simulink model "copia 15_10_26"  (R2026a)
settings: Solver=VariableStepAuto  StopTime=10  RelTol=1e-2  AbsTol=1e-2  EnableMultiTasking=on
values from neighbouring files (symbols this model uses):
  effective_bulkmodulus = 750e6    (= 750000000)    [MARLUP_hydr_params.m]
  m_load = 20    [MARLUP_hydr_params.m]
  p_supply = 160e5    (= 16000000)    [MARLUP_hydr_params.m]
  p_tank = 1.01325e5    (= 101325)    [MARLUP_hydr_params.m]
undefined symbols (not defined in the file or in its folder): cyl, Kd_heave, Kd_pitch, Kd_roll, Ki_heave, Ki_pitch, Ki_roll, Kp_heave, Kp_pitch, Kp_roll, pipe, Tinv, Ts, valve, X, Y, Z
libraries: sm_lib x75, nesl_utility x14, slpidlib x6, simulink x3
(part 5 of 5)

== system copia 15_10_26/PLANTA/Actuador_Hidraulico_2/cylinder_63_36/volume A chamber ==
  note: ∆𝑉 = −𝑉0 / 𝐵𝑛 ∗ ∆𝑝
  Q_in : Inport
  " dV/dt" : Inport  Port=2
  " V" : Inport  Port=3
  " B" : Inport  Port=4
  Integrator : Integrator  InitialCondition=cyl.p0A  AbsoluteTolerance=10
  Product : Product  Inputs=*/*  InputSameDT=on  SaturateOnIntegerOverflow=on  OutDataTypeStr=Inherit: Same as first input
  Saturation : Saturate  UpperLimit=inf  LowerLimit=-1e5
  Sum1 : Sum  Inputs=+-  InputSameDT=on  SaturateOnIntegerOverflow=on  OutDataTypeStr=Inherit: Same as first input
  p : Outport  VectorParamsAs1DForOutWhenUnconnected=off
  wires:
  Integrator/1 -> Saturation/1
  Product/1 -> Integrator/1
  Sum1/1 -> Product/1
  " B"/1 -> Product/3
  Saturation/1 -> p/1
  Q_in/1 -> Sum1/1
  " V"/1 -> Product/2
  " dV/dt"/1 -> Sum1/2

== system copia 15_10_26/PLANTA/Actuador_Hidraulico_2/cylinder_63_36/volume B chamber ==
  Q_in : Inport
  " dV/dt" : Inport  Port=2
  " V" : Inport  Port=3
  " B" : Inport  Port=4
  Integrator : Integrator  InitialCondition=cyl.p0B  AbsoluteTolerance=10
  Product : Product  Inputs=*/*  InputSameDT=on  SaturateOnIntegerOverflow=on  OutDataTypeStr=Inherit: Same as first input
  Saturation : Saturate  UpperLimit=inf  LowerLimit=-1e5
  Sum1 : Sum  Inputs=+-  InputSameDT=on  SaturateOnIntegerOverflow=on  OutDataTypeStr=Inherit: Same as first input
  p : Outport  VectorParamsAs1DForOutWhenUnconnected=off
  wires:
  " dV/dt"/1 -> Sum1/2
  " V"/1 -> Product/2
  Q_in/1 -> Sum1/1
  Saturation/1 -> p/1
  " B"/1 -> Product/3
  Sum1/1 -> Product/1
  Product/1 -> Integrator/1
  Integrator/1 -> Saturation/1

== system copia 15_10_26/PLANTA/Actuador_Hidraulico_2/gate_load_mass/load_fric ==
  v : Inport
  Gain1 : Gain  Gain=-1
  Product : Product  Inputs=4
  Sign : Signum
  coeff_fric : Constant  Value=0.7e5
  F_fric_load : Outport  VectorParamsAs1DForOutWhenUnconnected=off
  wires:
  Product/1 -> F_fric_load/1
  Sign/1 -> Gain1/1
  coeff_fric/1 -> Product/4
  Gain1/1 -> Product/1
  v/1 -> Product/2, Product/3, Sign/1

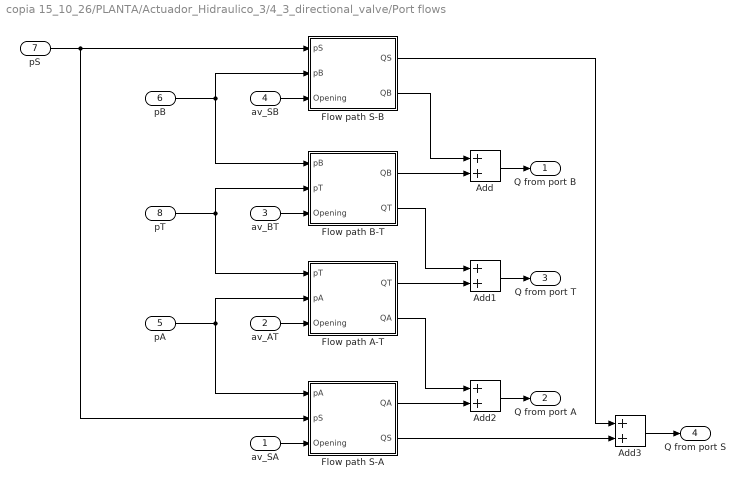
== system copia 15_10_26/PLANTA/Actuador_Hidraulico_3/4_3_directional_valve/Port flows ==
  av_SA : Inport
  av_AT : Inport  Port=2
  av_BT : Inport  Port=3
  av_SB : Inport  Port=4
  pA : Inport  Port=5
  pB : Inport  Port=6
  pS : Inport  Port=7
  pT : Inport  Port=8
  Add{,1..3} (4 alike) : Sum
  Flow path A-T : Subsystem  mask(Hydraulic){DPN=valve.dpN, QN=valve.QN, ptr=valve.ptr}
      mask prompts: DPN "Nominal Pressure Difference [Pa] :"; QN "Flow at nominal pressure difference and maximum opening [m^3/s] :"; ptr "Transition pressure [Pa] :"
      mask help:
      | Implements numerically robust turbulent flow equation. Polynomial flow equation is
      | used when abs(dp) is smaller than transition pressure.
      | [Source: Ellman, A. & Piche, R. 1996.
      | A Modified Orifice Flow Formula for Numerical Simulation of Fluid Power Systems.
      | Fluid Power Systems and Technology, ASME]
      mask init:
      | K = QN/(sqrt(DPN));
  Flow path B-T : Subsystem  mask(Hydraulic){DPN=valve.dpN, QN=valve.QN, ptr=valve.ptr}
      mask prompts: DPN "Nominal Pressure Difference [Pa] :"; QN "Flow at nominal pressure difference and maximum opening [m^3/s] :"; ptr "Transition pressure [Pa] :"
      mask help:
      | Implements numerically robust turbulent flow equation. Polynomial flow equation is
      | used when abs(dp) is smaller than transition pressure.
      | [Source: Ellman, A. & Piche, R. 1996.
      | A Modified Orifice Flow Formula for Numerical Simulation of Fluid Power Systems.
      | Fluid Power Systems and Technology, ASME]
      mask init:
      | K = QN/(sqrt(DPN));
  Flow path S-A : Subsystem  mask(Hydraulic){DPN=valve.dpN, QN=valve.QN, ptr=valve.ptr}
      mask prompts: DPN "Nominal Pressure Difference [Pa] :"; QN "Flow at nominal pressure difference and maximum opening [m^3/s] :"; ptr "Transition pressure [Pa] :"
      mask help:
      | Implements numerically robust turbulent flow equation. Polynomial flow equation is
      | used when abs(dp) is smaller than transition pressure.
      | [Source: Ellman, A. & Piche, R. 1996.
      | A Modified Orifice Flow Formula for Numerical Simulation of Fluid Power Systems.
      | Fluid Power Systems and Technology, ASME]
      mask init:
      | K = QN/(sqrt(DPN));
  Flow path S-B : Subsystem  mask(Hydraulic){DPN=valve.dpN, QN=valve.QN, ptr=valve.ptr}
      mask prompts: DPN "Nominal Pressure Difference [Pa] :"; QN "Flow at nominal pressure difference and maximum opening [m^3/s] :"; ptr "Transition pressure [Pa] :"
      mask help:
      | Implements numerically robust turbulent flow equation. Polynomial flow equation is
      | used when abs(dp) is smaller than transition pressure.
      | [Source: Ellman, A. & Piche, R. 1996.
      | A Modified Orifice Flow Formula for Numerical Simulation of Fluid Power Systems.
      | Fluid Power Systems and Technology, ASME]
      mask init:
      | K = QN/(sqrt(DPN));
  Q from port B : Outport  VectorParamsAs1DForOutWhenUnconnected=off
  Q from port A : Outport  Port=2  VectorParamsAs1DForOutWhenUnconnected=off
  Q from port T : Outport  Port=3  VectorParamsAs1DForOutWhenUnconnected=off
  Q from port S : Outport  Port=4  VectorParamsAs1DForOutWhenUnconnected=off
  wires:
  av_SA/1 -> Flow path S-A/3(Opening)
  av_AT/1 -> Flow path A-T/3(Opening)
  av_BT/1 -> Flow path B-T/3(Opening)
  pA/1 -> Flow path A-T/2(pA), Flow path S-A/1(pA)
  pB/1 -> Flow path B-T/1(pB), Flow path S-B/2(pB)
  pS/1 -> Flow path S-B/1(pS), Flow path S-A/2(pS)
  pT/1 -> Flow path A-T/1(pT), Flow path B-T/2(pT)
  Add/1 -> Q from port B/1
  Add1/1 -> Q from port T/1
  Add2/1 -> Q from port A/1
  Add3/1 -> Q from port S/1
  Flow path S-B/1(QS) -> Add3/1
  Flow path S-A/2(QS) -> Add3/2
  Flow path S-A/1(QA) -> Add2/2
  Flow path A-T/2(QA) -> Add2/1
  Flow path A-T/1(QT) -> Add1/2
  Flow path B-T/2(QT) -> Add1/1
  Flow path B-T/1(QB) -> Add/2
  Flow path S-B/2(QB) -> Add/1
  av_SB/1 -> Flow path S-B/3(Opening)

== system copia 15_10_26/PLANTA/Actuador_Hidraulico_3/4_3_directional_valve/Relative opening of flow paths ==
  x : Inport
  Gain : Gain  Gain=-1
  Lookup Table5 : Lookup  InputValues=[0.01 0.05 0.1 0.2 0.3 0.4 1]  Table=[0.01 0.039 0.078 0.16 0.23 0.31 0.78]  SaturateOnIntegerOverflow=off
  Lookup Table6 : Lookup  InputValues=[0.01 0.05 0.1 0.2 0.3 0.4 1]  Table=[0.01 0.036 0.072 0.14 0.22 0.29 0.72]  SaturateOnIntegerOverflow=off
  Lookup Table7 : Lookup  InputValues=[0.01 0.05 0.1 0.2 0.3 0.4 1]  Table=[0.01 0.039 0.077 0.15 0.23 0.31 0.77]  SaturateOnIntegerOverflow=off
  Lookup Table8 : Lookup  InputValues=[0.01 0.05 0.1 0.2 0.3 0.4 1]  Table=[0.01 0.035 0.070 0.14 0.21 0.28 0.70]  SaturateOnIntegerOverflow=off
  Saturation1 : Saturate  UpperLimit=1  LowerLimit=0
  Saturation2 : Saturate  UpperLimit=0  LowerLimit=-1
  av_SA : Outport  VectorParamsAs1DForOutWhenUnconnected=off
  av_AT : Outport  Port=2  VectorParamsAs1DForOutWhenUnconnected=off
  av_BT : Outport  Port=3  VectorParamsAs1DForOutWhenUnconnected=off
  av_SB : Outport  Port=4  VectorParamsAs1DForOutWhenUnconnected=off
  wires:
  x/1 -> Saturation2/1, Saturation1/1
  Saturation2/1 -> Gain/1
  Lookup Table8/1 -> av_AT/1
  Lookup Table7/1 -> av_SB/1
  Lookup Table6/1 -> av_BT/1
  Lookup Table5/1 -> av_SA/1
  Saturation1/1 -> Lookup Table5/1, Lookup Table6/1
  Gain/1 -> Lookup Table8/1, Lookup Table7/1

== system copia 15_10_26/PLANTA/Actuador_Hidraulico_3/4_3_directional_valve/Valve dynamics ==
  u : Inport
  Rate Limiter : RateLimiter  RisingSlewLimit=valve.ratelimit  FallingSlewLimit=-valve.ratelimit  SampleTimeMode=inherited
  Saturation limits [-1,1] : Saturate  UpperLimit=1  LowerLimit=-1
  Saturation limits [-1,1]2 : Saturate  UpperLimit=1  LowerLimit=-1
  Transfer Fcn1 : TransferFcn  Denominator=[valve.tau 1]
  Transport Delay of the valve : TransportDelay  DelayTime=valve.delay
  x : Outport  VectorParamsAs1DForOutWhenUnconnected=off
  wires:
  Saturation limits [-1,1]/1 -> Transport Delay of the valve/1
  Transport Delay of the valve/1 -> Rate Limiter/1
  Rate Limiter/1 -> Transfer Fcn1/1
  u/1 -> Saturation limits [-1,1]/1
  Transfer Fcn1/1 -> Saturation limits [-1,1]2/1
  Saturation limits [-1,1]2/1 -> x/1

== system copia 15_10_26/PLANTA/Actuador_Hidraulico_3/cylinder_63_36/A-chamber and pipe size submodel ==
  x_cyl : Inport
  A : Gain  Gain=pipe.area
  A chamber dead volume : Constant  Value=cyl.V0A
  Add : Sum  Inputs=+++
  Gain : Gain  Gain=cyl.A_piston
  Lenght : Constant  Value=pipe.lenght
  V : Outport  VectorParamsAs1DForOutWhenUnconnected=off
  wires:
  A/1 -> Add/3
  Lenght/1 -> A/1
  A chamber dead volume/1 -> Add/2
  Gain/1 -> Add/1
  x_cyl/1 -> Gain/1
  Add/1 -> V/1

== system copia 15_10_26/PLANTA/Actuador_Hidraulico_3/cylinder_63_36/B-chamber and pipe size submodel ==
  x_cyl : Inport
  A : Gain  Gain=pipe.area
  Add : Sum  Inputs=+-
  Add1 : Sum  Inputs=+++
  B chamber dead volume : Constant  Value=cyl.V0B
  Cylinder stroke : Constant  Value=cyl.stroke
  Gain1 : Gain  Gain=cyl.A_rodside
  Lenght : Constant  Value=pipe.lenght
  V : Outport  VectorParamsAs1DForOutWhenUnconnected=off
  wires:
  A/1 -> Add1/3
  Lenght/1 -> A/1
  Cylinder stroke/1 -> Add/1
  Gain1/1 -> Add1/1
  Add/1 -> Gain1/1
  x_cyl/1 -> Add/2
  B chamber dead volume/1 -> Add1/2
  Add1/1 -> V/1

== system copia 15_10_26/PLANTA/Actuador_Hidraulico_3/cylinder_63_36/dynamic_fric_limited ==
  v : Inport
  Abs : Abs  SaturateOnIntegerOverflow=off
  Product : Product
  Sign : Signum
  cyl_fric_up_to_100mm/s : Lookup_n-D  NumberOfTableDimensions=1  BreakpointsForDimension1=|  Table=|  InternalRulePriority=Speed  RndMeth=Simplest
      BreakpointsForDimension1=|
      | [0
      | 5
      | 10
      | 15
      | 20
      | 25
      | 30
      | 35
      | 40
      | 45
      | 50
      | 55
      | 60
      | 65
      | 70
      | 75
      | 80
      | 85
      | 90
      | 95
      | 100]./1e3;
      Table=|
      | [0
      | 242
      | 550
      | 838
      | 996
      | 972
      | 850
      | 757
      | 728
      | 733
      | 744
      | 753
      | 759
      | 765
      | 770
      | 775
      | 780
      | 785
      | 790
      | 795
      | 800];
  F_fric : Outport  VectorParamsAs1DForOutWhenUnconnected=off
  wires:
  Abs/1 -> cyl_fric_up_to_100mm/s/1
  v/1 -> Sign/1, Abs/1
  cyl_fric_up_to_100mm/s/1 -> Product/1
  Sign/1 -> Product/2
  Product/1 -> F_fric/1

== system copia 15_10_26/PLANTA/Actuador_Hidraulico_3/cylinder_63_36/volume A chamber ==
  note: ∆𝑉 = −𝑉0 / 𝐵𝑛 ∗ ∆𝑝
  Q_in : Inport
  " dV/dt" : Inport  Port=2
  " V" : Inport  Port=3
  " B" : Inport  Port=4
  Integrator : Integrator  InitialCondition=cyl.p0A  AbsoluteTolerance=10
  Product : Product  Inputs=*/*  InputSameDT=on  SaturateOnIntegerOverflow=on  OutDataTypeStr=Inherit: Same as first input
  Saturation : Saturate  UpperLimit=inf  LowerLimit=-1e5
  Sum1 : Sum  Inputs=+-  InputSameDT=on  SaturateOnIntegerOverflow=on  OutDataTypeStr=Inherit: Same as first input
  p : Outport  VectorParamsAs1DForOutWhenUnconnected=off
  wires:
  Integrator/1 -> Saturation/1
  Product/1 -> Integrator/1
  Sum1/1 -> Product/1
  " B"/1 -> Product/3
  Saturation/1 -> p/1
  Q_in/1 -> Sum1/1
  " V"/1 -> Product/2
  " dV/dt"/1 -> Sum1/2

== system copia 15_10_26/PLANTA/Actuador_Hidraulico_3/cylinder_63_36/volume B chamber ==
  Q_in : Inport
  " dV/dt" : Inport  Port=2
  " V" : Inport  Port=3
  " B" : Inport  Port=4
  Integrator : Integrator  InitialCondition=cyl.p0B  AbsoluteTolerance=10
  Product : Product  Inputs=*/*  InputSameDT=on  SaturateOnIntegerOverflow=on  OutDataTypeStr=Inherit: Same as first input
  Saturation : Saturate  UpperLimit=inf  LowerLimit=-1e5
  Sum1 : Sum  Inputs=+-  InputSameDT=on  SaturateOnIntegerOverflow=on  OutDataTypeStr=Inherit: Same as first input
  p : Outport  VectorParamsAs1DForOutWhenUnconnected=off
  wires:
  " dV/dt"/1 -> Sum1/2
  " V"/1 -> Product/2
  Q_in/1 -> Sum1/1
  Saturation/1 -> p/1
  " B"/1 -> Product/3
  Sum1/1 -> Product/1
  Product/1 -> Integrator/1
  Integrator/1 -> Saturation/1

== system copia 15_10_26/PLANTA/Actuador_Hidraulico_3/gate_load_mass/load_fric ==
  v : Inport
  Gain1 : Gain  Gain=-1
  Product : Product  Inputs=4
  Sign : Signum
  coeff_fric : Constant  Value=0.7e5
  F_fric_load : Outport  VectorParamsAs1DForOutWhenUnconnected=off
  wires:
  Product/1 -> F_fric_load/1
  Sign/1 -> Gain1/1
  coeff_fric/1 -> Product/4
  Gain1/1 -> Product/1
  v/1 -> Product/2, Product/3, Sign/1

== system copia 15_10_26/PLANTA/Actuador_Hidraulico_1/4_3_directional_valve/Port flows/Flow path A-T ==
  pT : Inport
  pA : Inport  Port=2
  Opening : Inport  Port=3
  Abs : Abs  ZeroCross=off
  Flow coefficient : Gain  Gain=K  SaturateOnIntegerOverflow=on  OutDataTypeStr=Inherit: Same as input  ParamDataTypeStr=Inherit: Same as input
  Gain1 : Gain  Gain=-1  SaturateOnIntegerOverflow=on  OutDataTypeStr=Inherit: Same as input  ParamDataTypeStr=Inherit: Same as input
  Limit opening to non-negative : Saturate  UpperLimit=inf  LowerLimit=0
  Math Function1 : Math  Operator=sqrt  SignedPower=on
  Mux : Mux  Inputs=2
  Polynomial flow equation : Fcn  Expr=u[2]*u[1]/2.0/sqrt(ptr)*(3-u[1]/ptr)
  Product : Product  InputSameDT=on  SaturateOnIntegerOverflow=on  OutDataTypeStr=Inherit: Same as first input
  Product1 : Product  InputSameDT=on  SaturateOnIntegerOverflow=on  OutDataTypeStr=Inherit: Same as first input
  Sign : Signum  ZeroCross=off
  Sum : Sum  Inputs=|+-
  Switch : Switch  Threshold=ptr  ZeroCross=off
  QT : Outport  InitialOutput=0  VectorParamsAs1DForOutWhenUnconnected=off
  QA : Outport  Port=2  InitialOutput=0  VectorParamsAs1DForOutWhenUnconnected=off
  wires:
  Opening/1 -> Limit opening to non-negative/1
  Sum/1 -> Abs/1, Sign/1
  Polynomial flow equation/1 -> Switch/3
  Mux/1 -> Polynomial flow equation/1
  Product/1 -> Switch/1
  Math Function1/1 -> Product/1
  Abs/1 -> Mux/1, Switch/2, Math Function1/1
  Limit opening to non-negative/1 -> Flow coefficient/1
  Flow coefficient/1 -> Product/2, Mux/2
  Sign/1 -> Product1/1
  Product1/1 -> Gain1/1, QT/1
  Switch/1 -> Product1/2
  pA/1 -> Sum/1
  pT/1 -> Sum/2
  Gain1/1 -> QA/1

== system copia 15_10_26/PLANTA/Actuador_Hidraulico_1/4_3_directional_valve/Port flows/Flow path B-T ==
  pB : Inport
  pT : Inport  Port=2
  Opening : Inport  Port=3
  Abs : Abs  ZeroCross=off
  Flow coefficient : Gain  Gain=K  SaturateOnIntegerOverflow=on  OutDataTypeStr=Inherit: Same as input  ParamDataTypeStr=Inherit: Same as input
  Gain1 : Gain  Gain=-1  SaturateOnIntegerOverflow=on  OutDataTypeStr=Inherit: Same as input  ParamDataTypeStr=Inherit: Same as input
  Limit opening to non-negative : Saturate  UpperLimit=inf  LowerLimit=0
  Math Function1 : Math  Operator=sqrt  SignedPower=on
  Mux : Mux  Inputs=2
  Polynomial flow equation : Fcn  Expr=u[2]*u[1]/2.0/sqrt(ptr)*(3-u[1]/ptr)
  Product : Product  InputSameDT=on  SaturateOnIntegerOverflow=on  OutDataTypeStr=Inherit: Same as first input
  Product1 : Product  InputSameDT=on  SaturateOnIntegerOverflow=on  OutDataTypeStr=Inherit: Same as first input
  Sign : Signum  ZeroCross=off
  Sum : Sum  Inputs=|+-
  Switch : Switch  Threshold=ptr  ZeroCross=off
  QB : Outport  InitialOutput=0  VectorParamsAs1DForOutWhenUnconnected=off
  QT : Outport  Port=2  InitialOutput=0  VectorParamsAs1DForOutWhenUnconnected=off
  wires:
  Gain1/1 -> QB/1
  pT/1 -> Sum/2
  pB/1 -> Sum/1
  Switch/1 -> Product1/2
  Product1/1 -> QT/1, Gain1/1
  Sign/1 -> Product1/1
  Flow coefficient/1 -> Mux/2, Product/2
  Limit opening to non-negative/1 -> Flow coefficient/1
  Abs/1 -> Math Function1/1, Switch/2, Mux/1
  Math Function1/1 -> Product/1
  Product/1 -> Switch/1
  Mux/1 -> Polynomial flow equation/1
  Polynomial flow equation/1 -> Switch/3
  Sum/1 -> Sign/1, Abs/1
  Opening/1 -> Limit opening to non-negative/1

== system copia 15_10_26/PLANTA/Actuador_Hidraulico_1/4_3_directional_valve/Port flows/Flow path S-A ==
  pA : Inport
  pS : Inport  Port=2
  Opening : Inport  Port=3
  Abs : Abs  ZeroCross=off
  Flow coefficient : Gain  Gain=K  SaturateOnIntegerOverflow=on  OutDataTypeStr=Inherit: Same as input  ParamDataTypeStr=Inherit: Same as input
  Gain1 : Gain  Gain=-1  SaturateOnIntegerOverflow=on  OutDataTypeStr=Inherit: Same as input  ParamDataTypeStr=Inherit: Same as input
  Limit opening to non-negative : Saturate  UpperLimit=inf  LowerLimit=0
  Math Function1 : Math  Operator=sqrt  SignedPower=on
  Mux : Mux  Inputs=2
  Polynomial flow equation : Fcn  Expr=u[2]*u[1]/2.0/sqrt(ptr)*(3-u[1]/ptr)
  Product : Product  InputSameDT=on  SaturateOnIntegerOverflow=on  OutDataTypeStr=Inherit: Same as first input
  Product1 : Product  InputSameDT=on  SaturateOnIntegerOverflow=on  OutDataTypeStr=Inherit: Same as first input
  Sign : Signum  ZeroCross=off
  Sum : Sum  Inputs=|+-
  Switch : Switch  Threshold=ptr  ZeroCross=off
  QA : Outport  InitialOutput=0  VectorParamsAs1DForOutWhenUnconnected=off
  QS : Outport  Port=2  InitialOutput=0  VectorParamsAs1DForOutWhenUnconnected=off
  wires:
  Opening/1 -> Limit opening to non-negative/1
  Sum/1 -> Abs/1, Sign/1
  Polynomial flow equation/1 -> Switch/3
  Mux/1 -> Polynomial flow equation/1
  Product/1 -> Switch/1
  Math Function1/1 -> Product/1
  Abs/1 -> Mux/1, Switch/2, Math Function1/1
  Limit opening to non-negative/1 -> Flow coefficient/1
  Flow coefficient/1 -> Product/2, Mux/2
  Sign/1 -> Product1/1
  Product1/1 -> Gain1/1, QA/1
  Switch/1 -> Product1/2
  pS/1 -> Sum/1
  pA/1 -> Sum/2
  Gain1/1 -> QS/1

== system copia 15_10_26/PLANTA/Actuador_Hidraulico_1/4_3_directional_valve/Port flows/Flow path S-B ==
  pS : Inport
  pB : Inport  Port=2
  Opening : Inport  Port=3
  Abs : Abs  ZeroCross=off
  Flow coefficient : Gain  Gain=K  SaturateOnIntegerOverflow=on  OutDataTypeStr=Inherit: Same as input  ParamDataTypeStr=Inherit: Same as input
  Gain1 : Gain  Gain=-1  SaturateOnIntegerOverflow=on  OutDataTypeStr=Inherit: Same as input  ParamDataTypeStr=Inherit: Same as input
  Limit opening to non-negative : Saturate  UpperLimit=inf  LowerLimit=0
  Math Function1 : Math  Operator=sqrt  SignedPower=on
  Mux : Mux  Inputs=2
  Polynomial flow equation : Fcn  Expr=u[2]*u[1]/2.0/sqrt(ptr)*(3-u[1]/ptr)
  Product : Product  InputSameDT=on  SaturateOnIntegerOverflow=on  OutDataTypeStr=Inherit: Same as first input
  Product1 : Product  InputSameDT=on  SaturateOnIntegerOverflow=on  OutDataTypeStr=Inherit: Same as first input
  Sign : Signum  ZeroCross=off
  Sum : Sum  Inputs=|+-
  Switch : Switch  Threshold=ptr  ZeroCross=off
  QS : Outport  InitialOutput=0  VectorParamsAs1DForOutWhenUnconnected=off
  QB : Outport  Port=2  InitialOutput=0  VectorParamsAs1DForOutWhenUnconnected=off
  wires:
  Gain1/1 -> QS/1
  pB/1 -> Sum/2
  pS/1 -> Sum/1
  Switch/1 -> Product1/2
  Product1/1 -> QB/1, Gain1/1
  Sign/1 -> Product1/1
  Flow coefficient/1 -> Mux/2, Product/2
  Limit opening to non-negative/1 -> Flow coefficient/1
  Abs/1 -> Math Function1/1, Switch/2, Mux/1
  Math Function1/1 -> Product/1
  Product/1 -> Switch/1
  Mux/1 -> Polynomial flow equation/1
  Polynomial flow equation/1 -> Switch/3
  Sum/1 -> Sign/1, Abs/1
  Opening/1 -> Limit opening to non-negative/1

== system copia 15_10_26/PLANTA/Actuador_Hidraulico_2/4_3_directional_valve/Port flows/Flow path A-T ==
  pT : Inport
  pA : Inport  Port=2
  Opening : Inport  Port=3
  Abs : Abs  ZeroCross=off
  Flow coefficient : Gain  Gain=K  SaturateOnIntegerOverflow=on  OutDataTypeStr=Inherit: Same as input  ParamDataTypeStr=Inherit: Same as input
  Gain1 : Gain  Gain=-1  SaturateOnIntegerOverflow=on  OutDataTypeStr=Inherit: Same as input  ParamDataTypeStr=Inherit: Same as input
  Limit opening to non-negative : Saturate  UpperLimit=inf  LowerLimit=0
  Math Function1 : Math  Operator=sqrt  SignedPower=on
  Mux : Mux  Inputs=2
  Polynomial flow equation : Fcn  Expr=u[2]*u[1]/2.0/sqrt(ptr)*(3-u[1]/ptr)
  Product : Product  InputSameDT=on  SaturateOnIntegerOverflow=on  OutDataTypeStr=Inherit: Same as first input
  Product1 : Product  InputSameDT=on  SaturateOnIntegerOverflow=on  OutDataTypeStr=Inherit: Same as first input
  Sign : Signum  ZeroCross=off
  Sum : Sum  Inputs=|+-
  Switch : Switch  Threshold=ptr  ZeroCross=off
  QT : Outport  InitialOutput=0  VectorParamsAs1DForOutWhenUnconnected=off
  QA : Outport  Port=2  InitialOutput=0  VectorParamsAs1DForOutWhenUnconnected=off
  wires:
  Opening/1 -> Limit opening to non-negative/1
  Sum/1 -> Abs/1, Sign/1
  Polynomial flow equation/1 -> Switch/3
  Mux/1 -> Polynomial flow equation/1
  Product/1 -> Switch/1
  Math Function1/1 -> Product/1
  Abs/1 -> Mux/1, Switch/2, Math Function1/1
  Limit opening to non-negative/1 -> Flow coefficient/1
  Flow coefficient/1 -> Product/2, Mux/2
  Sign/1 -> Product1/1
  Product1/1 -> Gain1/1, QT/1
  Switch/1 -> Product1/2
  pA/1 -> Sum/1
  pT/1 -> Sum/2
  Gain1/1 -> QA/1

== system copia 15_10_26/PLANTA/Actuador_Hidraulico_2/4_3_directional_valve/Port flows/Flow path B-T ==
  pB : Inport
  pT : Inport  Port=2
  Opening : Inport  Port=3
  Abs : Abs  ZeroCross=off
  Flow coefficient : Gain  Gain=K  SaturateOnIntegerOverflow=on  OutDataTypeStr=Inherit: Same as input  ParamDataTypeStr=Inherit: Same as input
  Gain1 : Gain  Gain=-1  SaturateOnIntegerOverflow=on  OutDataTypeStr=Inherit: Same as input  ParamDataTypeStr=Inherit: Same as input
  Limit opening to non-negative : Saturate  UpperLimit=inf  LowerLimit=0
  Math Function1 : Math  Operator=sqrt  SignedPower=on
  Mux : Mux  Inputs=2
  Polynomial flow equation : Fcn  Expr=u[2]*u[1]/2.0/sqrt(ptr)*(3-u[1]/ptr)
  Product : Product  InputSameDT=on  SaturateOnIntegerOverflow=on  OutDataTypeStr=Inherit: Same as first input
  Product1 : Product  InputSameDT=on  SaturateOnIntegerOverflow=on  OutDataTypeStr=Inherit: Same as first input
  Sign : Signum  ZeroCross=off
  Sum : Sum  Inputs=|+-
  Switch : Switch  Threshold=ptr  ZeroCross=off
  QB : Outport  InitialOutput=0  VectorParamsAs1DForOutWhenUnconnected=off
  QT : Outport  Port=2  InitialOutput=0  VectorParamsAs1DForOutWhenUnconnected=off
  wires:
  Gain1/1 -> QB/1
  pT/1 -> Sum/2
  pB/1 -> Sum/1
  Switch/1 -> Product1/2
  Product1/1 -> QT/1, Gain1/1
  Sign/1 -> Product1/1
  Flow coefficient/1 -> Mux/2, Product/2
  Limit opening to non-negative/1 -> Flow coefficient/1
  Abs/1 -> Math Function1/1, Switch/2, Mux/1
  Math Function1/1 -> Product/1
  Product/1 -> Switch/1
  Mux/1 -> Polynomial flow equation/1
  Polynomial flow equation/1 -> Switch/3
  Sum/1 -> Sign/1, Abs/1
  Opening/1 -> Limit opening to non-negative/1

== system copia 15_10_26/PLANTA/Actuador_Hidraulico_2/4_3_directional_valve/Port flows/Flow path S-A ==
  pA : Inport
  pS : Inport  Port=2
  Opening : Inport  Port=3
  Abs : Abs  ZeroCross=off
  Flow coefficient : Gain  Gain=K  SaturateOnIntegerOverflow=on  OutDataTypeStr=Inherit: Same as input  ParamDataTypeStr=Inherit: Same as input
  Gain1 : Gain  Gain=-1  SaturateOnIntegerOverflow=on  OutDataTypeStr=Inherit: Same as input  ParamDataTypeStr=Inherit: Same as input
  Limit opening to non-negative : Saturate  UpperLimit=inf  LowerLimit=0
  Math Function1 : Math  Operator=sqrt  SignedPower=on
  Mux : Mux  Inputs=2
  Polynomial flow equation : Fcn  Expr=u[2]*u[1]/2.0/sqrt(ptr)*(3-u[1]/ptr)
  Product : Product  InputSameDT=on  SaturateOnIntegerOverflow=on  OutDataTypeStr=Inherit: Same as first input
  Product1 : Product  InputSameDT=on  SaturateOnIntegerOverflow=on  OutDataTypeStr=Inherit: Same as first input
  Sign : Signum  ZeroCross=off
  Sum : Sum  Inputs=|+-
  Switch : Switch  Threshold=ptr  ZeroCross=off
  QA : Outport  InitialOutput=0  VectorParamsAs1DForOutWhenUnconnected=off
  QS : Outport  Port=2  InitialOutput=0  VectorParamsAs1DForOutWhenUnconnected=off
  wires:
  Opening/1 -> Limit opening to non-negative/1
  Sum/1 -> Abs/1, Sign/1
  Polynomial flow equation/1 -> Switch/3
  Mux/1 -> Polynomial flow equation/1
  Product/1 -> Switch/1
  Math Function1/1 -> Product/1
  Abs/1 -> Mux/1, Switch/2, Math Function1/1
  Limit opening to non-negative/1 -> Flow coefficient/1
  Flow coefficient/1 -> Product/2, Mux/2
  Sign/1 -> Product1/1
  Product1/1 -> Gain1/1, QA/1
  Switch/1 -> Product1/2
  pS/1 -> Sum/1
  pA/1 -> Sum/2
  Gain1/1 -> QS/1

== system copia 15_10_26/PLANTA/Actuador_Hidraulico_2/4_3_directional_valve/Port flows/Flow path S-B ==
  pS : Inport
  pB : Inport  Port=2
  Opening : Inport  Port=3
  Abs : Abs  ZeroCross=off
  Flow coefficient : Gain  Gain=K  SaturateOnIntegerOverflow=on  OutDataTypeStr=Inherit: Same as input  ParamDataTypeStr=Inherit: Same as input
  Gain1 : Gain  Gain=-1  SaturateOnIntegerOverflow=on  OutDataTypeStr=Inherit: Same as input  ParamDataTypeStr=Inherit: Same as input
  Limit opening to non-negative : Saturate  UpperLimit=inf  LowerLimit=0
  Math Function1 : Math  Operator=sqrt  SignedPower=on
  Mux : Mux  Inputs=2
  Polynomial flow equation : Fcn  Expr=u[2]*u[1]/2.0/sqrt(ptr)*(3-u[1]/ptr)
  Product : Product  InputSameDT=on  SaturateOnIntegerOverflow=on  OutDataTypeStr=Inherit: Same as first input
  Product1 : Product  InputSameDT=on  SaturateOnIntegerOverflow=on  OutDataTypeStr=Inherit: Same as first input
  Sign : Signum  ZeroCross=off
  Sum : Sum  Inputs=|+-
  Switch : Switch  Threshold=ptr  ZeroCross=off
  QS : Outport  InitialOutput=0  VectorParamsAs1DForOutWhenUnconnected=off
  QB : Outport  Port=2  InitialOutput=0  VectorParamsAs1DForOutWhenUnconnected=off
  wires:
  Gain1/1 -> QS/1
  pB/1 -> Sum/2
  pS/1 -> Sum/1
  Switch/1 -> Product1/2
  Product1/1 -> QB/1, Gain1/1
  Sign/1 -> Product1/1
  Flow coefficient/1 -> Mux/2, Product/2
  Limit opening to non-negative/1 -> Flow coefficient/1
  Abs/1 -> Math Function1/1, Switch/2, Mux/1
  Math Function1/1 -> Product/1
  Product/1 -> Switch/1
  Mux/1 -> Polynomial flow equation/1
  Polynomial flow equation/1 -> Switch/3
  Sum/1 -> Sign/1, Abs/1
  Opening/1 -> Limit opening to non-negative/1

== system copia 15_10_26/PLANTA/Actuador_Hidraulico_3/4_3_directional_valve/Port flows/Flow path A-T ==
  pT : Inport
  pA : Inport  Port=2
  Opening : Inport  Port=3
  Abs : Abs  ZeroCross=off
  Flow coefficient : Gain  Gain=K  SaturateOnIntegerOverflow=on  OutDataTypeStr=Inherit: Same as input  ParamDataTypeStr=Inherit: Same as input
  Gain1 : Gain  Gain=-1  SaturateOnIntegerOverflow=on  OutDataTypeStr=Inherit: Same as input  ParamDataTypeStr=Inherit: Same as input
  Limit opening to non-negative : Saturate  UpperLimit=inf  LowerLimit=0
  Math Function1 : Math  Operator=sqrt  SignedPower=on
  Mux : Mux  Inputs=2
  Polynomial flow equation : Fcn  Expr=u[2]*u[1]/2.0/sqrt(ptr)*(3-u[1]/ptr)
  Product : Product  InputSameDT=on  SaturateOnIntegerOverflow=on  OutDataTypeStr=Inherit: Same as first input
  Product1 : Product  InputSameDT=on  SaturateOnIntegerOverflow=on  OutDataTypeStr=Inherit: Same as first input
  Sign : Signum  ZeroCross=off
  Sum : Sum  Inputs=|+-
  Switch : Switch  Threshold=ptr  ZeroCross=off
  QT : Outport  InitialOutput=0  VectorParamsAs1DForOutWhenUnconnected=off
  QA : Outport  Port=2  InitialOutput=0  VectorParamsAs1DForOutWhenUnconnected=off
  wires:
  Opening/1 -> Limit opening to non-negative/1
  Sum/1 -> Abs/1, Sign/1
  Polynomial flow equation/1 -> Switch/3
  Mux/1 -> Polynomial flow equation/1
  Product/1 -> Switch/1
  Math Function1/1 -> Product/1
  Abs/1 -> Mux/1, Switch/2, Math Function1/1
  Limit opening to non-negative/1 -> Flow coefficient/1
  Flow coefficient/1 -> Product/2, Mux/2
  Sign/1 -> Product1/1
  Product1/1 -> Gain1/1, QT/1
  Switch/1 -> Product1/2
  pA/1 -> Sum/1
  pT/1 -> Sum/2
  Gain1/1 -> QA/1

== system copia 15_10_26/PLANTA/Actuador_Hidraulico_3/4_3_directional_valve/Port flows/Flow path B-T ==
  pB : Inport
  pT : Inport  Port=2
  Opening : Inport  Port=3
  Abs : Abs  ZeroCross=off
  Flow coefficient : Gain  Gain=K  SaturateOnIntegerOverflow=on  OutDataTypeStr=Inherit: Same as input  ParamDataTypeStr=Inherit: Same as input
  Gain1 : Gain  Gain=-1  SaturateOnIntegerOverflow=on  OutDataTypeStr=Inherit: Same as input  ParamDataTypeStr=Inherit: Same as input
  Limit opening to non-negative : Saturate  UpperLimit=inf  LowerLimit=0
  Math Function1 : Math  Operator=sqrt  SignedPower=on
  Mux : Mux  Inputs=2
  Polynomial flow equation : Fcn  Expr=u[2]*u[1]/2.0/sqrt(ptr)*(3-u[1]/ptr)
  Product : Product  InputSameDT=on  SaturateOnIntegerOverflow=on  OutDataTypeStr=Inherit: Same as first input
  Product1 : Product  InputSameDT=on  SaturateOnIntegerOverflow=on  OutDataTypeStr=Inherit: Same as first input
  Sign : Signum  ZeroCross=off
  Sum : Sum  Inputs=|+-
  Switch : Switch  Threshold=ptr  ZeroCross=off
  QB : Outport  InitialOutput=0  VectorParamsAs1DForOutWhenUnconnected=off
  QT : Outport  Port=2  InitialOutput=0  VectorParamsAs1DForOutWhenUnconnected=off
  wires:
  Gain1/1 -> QB/1
  pT/1 -> Sum/2
  pB/1 -> Sum/1
  Switch/1 -> Product1/2
  Product1/1 -> QT/1, Gain1/1
  Sign/1 -> Product1/1
  Flow coefficient/1 -> Mux/2, Product/2
  Limit opening to non-negative/1 -> Flow coefficient/1
  Abs/1 -> Math Function1/1, Switch/2, Mux/1
  Math Function1/1 -> Product/1
  Product/1 -> Switch/1
  Mux/1 -> Polynomial flow equation/1
  Polynomial flow equation/1 -> Switch/3
  Sum/1 -> Sign/1, Abs/1
  Opening/1 -> Limit opening to non-negative/1

== system copia 15_10_26/PLANTA/Actuador_Hidraulico_3/4_3_directional_valve/Port flows/Flow path S-A ==
  pA : Inport
  pS : Inport  Port=2
  Opening : Inport  Port=3
  Abs : Abs  ZeroCross=off
  Flow coefficient : Gain  Gain=K  SaturateOnIntegerOverflow=on  OutDataTypeStr=Inherit: Same as input  ParamDataTypeStr=Inherit: Same as input
  Gain1 : Gain  Gain=-1  SaturateOnIntegerOverflow=on  OutDataTypeStr=Inherit: Same as input  ParamDataTypeStr=Inherit: Same as input
  Limit opening to non-negative : Saturate  UpperLimit=inf  LowerLimit=0
  Math Function1 : Math  Operator=sqrt  SignedPower=on
  Mux : Mux  Inputs=2
  Polynomial flow equation : Fcn  Expr=u[2]*u[1]/2.0/sqrt(ptr)*(3-u[1]/ptr)
  Product : Product  InputSameDT=on  SaturateOnIntegerOverflow=on  OutDataTypeStr=Inherit: Same as first input
  Product1 : Product  InputSameDT=on  SaturateOnIntegerOverflow=on  OutDataTypeStr=Inherit: Same as first input
  Sign : Signum  ZeroCross=off
  Sum : Sum  Inputs=|+-
  Switch : Switch  Threshold=ptr  ZeroCross=off
  QA : Outport  InitialOutput=0  VectorParamsAs1DForOutWhenUnconnected=off
  QS : Outport  Port=2  InitialOutput=0  VectorParamsAs1DForOutWhenUnconnected=off
  wires:
  Opening/1 -> Limit opening to non-negative/1
  Sum/1 -> Abs/1, Sign/1
  Polynomial flow equation/1 -> Switch/3
  Mux/1 -> Polynomial flow equation/1
  Product/1 -> Switch/1
  Math Function1/1 -> Product/1
  Abs/1 -> Mux/1, Switch/2, Math Function1/1
  Limit opening to non-negative/1 -> Flow coefficient/1
  Flow coefficient/1 -> Product/2, Mux/2
  Sign/1 -> Product1/1
  Product1/1 -> Gain1/1, QA/1
  Switch/1 -> Product1/2
  pS/1 -> Sum/1
  pA/1 -> Sum/2
  Gain1/1 -> QS/1

== system copia 15_10_26/PLANTA/Actuador_Hidraulico_3/4_3_directional_valve/Port flows/Flow path S-B ==
  pS : Inport
  pB : Inport  Port=2
  Opening : Inport  Port=3
  Abs : Abs  ZeroCross=off
  Flow coefficient : Gain  Gain=K  SaturateOnIntegerOverflow=on  OutDataTypeStr=Inherit: Same as input  ParamDataTypeStr=Inherit: Same as input
  Gain1 : Gain  Gain=-1  SaturateOnIntegerOverflow=on  OutDataTypeStr=Inherit: Same as input  ParamDataTypeStr=Inherit: Same as input
  Limit opening to non-negative : Saturate  UpperLimit=inf  LowerLimit=0
  Math Function1 : Math  Operator=sqrt  SignedPower=on
  Mux : Mux  Inputs=2
  Polynomial flow equation : Fcn  Expr=u[2]*u[1]/2.0/sqrt(ptr)*(3-u[1]/ptr)
  Product : Product  InputSameDT=on  SaturateOnIntegerOverflow=on  OutDataTypeStr=Inherit: Same as first input
  Product1 : Product  InputSameDT=on  SaturateOnIntegerOverflow=on  OutDataTypeStr=Inherit: Same as first input
  Sign : Signum  ZeroCross=off
  Sum : Sum  Inputs=|+-
  Switch : Switch  Threshold=ptr  ZeroCross=off
  QS : Outport  InitialOutput=0  VectorParamsAs1DForOutWhenUnconnected=off
  QB : Outport  Port=2  InitialOutput=0  VectorParamsAs1DForOutWhenUnconnected=off
  wires:
  Gain1/1 -> QS/1
  pB/1 -> Sum/2
  pS/1 -> Sum/1
  Switch/1 -> Product1/2
  Product1/1 -> QB/1, Gain1/1
  Sign/1 -> Product1/1
  Flow coefficient/1 -> Mux/2, Product/2
  Limit opening to non-negative/1 -> Flow coefficient/1
  Abs/1 -> Math Function1/1, Switch/2, Mux/1
  Math Function1/1 -> Product/1
  Product/1 -> Switch/1
  Mux/1 -> Polynomial flow equation/1
  Polynomial flow equation/1 -> Switch/3
  Sum/1 -> Sign/1, Abs/1
  Opening/1 -> Limit opening to non-negative/1

== matlab function copia 15_10_26/PLANTA/P-M SPECTRUM/P-M SPECTRUM ==
  settings: updateMethod=DISCRETE
  data: t input; heave output; Hs input; Tp input; pitch output; roll output
function [heave, pitch, roll] = fcn(t, Hs, Tp)
%#codegen
% Esta función genera la elevación (heave), y los ángulos de inclinación 
% (pitch y roll) en el origen (0,0) para un oleaje P-M.
%
% Se utiliza t==0 para una inicialización robusta.

% -- Declaración de variables persistentes --
% Estas variables retienen su valor entre llamadas a la función.
persistent Anm fase omega kx ky

% -- Bloque de Inicialización --
% Este código se ejecuta UNA SOLA VEZ, al puro inicio de la simulación (t=0).
if t == 0
    
    % Parámetros fijos de la simulación
    N = 100;         % Número de componentes de frecuencia
    M = 50;          % Número de componentes de dirección
    g = 9.81;        % Aceleración de la gravedad

    % --- PRE-CÁLCULOS (se ejecutan solo una vez) ---
    fp = 1 / Tp;
    f_max = 4 * fp;
    df = f_max / N;
    f = df:df:f_max;
    omega = 2 * pi * f;

    d_theta = 2*pi / M;
    theta = d_theta:d_theta:2*pi;
    
    % Semilla fija: el mismo estado de mar en cada corrida, para poder
    % comparar controladores y reproducir resultados.
    rng(42);

    % Generar fases aleatorias (fijas para toda la simulación)
    fase = 2 * pi * rand(N, M);

    k_o = omega.^2 / g;
    kx = k_o' * cos(theta);
    ky = k_o' * sin(theta);
    
    A_pm = (5/16) * Hs^2 * fp^4;
    S = (A_pm ./ f.^5) .* exp(-1.25 * (fp^4 ./ f.^4));

    s = 10;
    D_theta = (2/pi) * (cos(theta/2)).^(2*s);
    D_theta(theta < -pi/2 | theta > pi/2) = 0;
    
    Anm = sqrt(2 * S' .* D_theta * df * d_theta);
end

% -- CÁLCULOS EN CADA PASO DE TIEMPO --
% Se requiere que las variables persistentes no estén vacías después de t=0
if isempty(Anm)
    % Si la inicialización no ha ocurrido (ej. si la simulación no empezó en t=0),
    % se asignan salidas cero para evitar errores.
    heave = 0;
    pitch = 0;
    roll = 0;
else
    % Cálculos normales para t > 0
    arg = -omega' * t + fase;
    heave = sum(Anm .* cos(arg), 'all');
    d_etadx = sum(Anm .* kx .* sin(arg), 'all');
    d_etady = sum(Anm .* ky .* sin(arg), 'all');
    pitch = atan(d_etadx);
    roll  = atan(d_etady);
end

end

== matlab function copia 15_10_26/PLANTA/INVERSE  KINEMATICS ==
  settings: updateMethod=DISCRETE
  data: dL output; alpha input; theta input; z input; L output; L0 output; R_TOP input
function [dL, L, L0] = marlup_ik(alpha, theta, z, R_TOP)
%MARLUP_IK  Cinematica inversa de MARLUP: (roll, pitch, heave) -> pistones.
%
%   [dL, L, L0] = MARLUP_IK(alpha, theta, z)
%
%   El calculo depende UNICAMENTE de la geometria de los anclajes:
%   radio inferior, radio superior y altura nominal entre soportes.
%   Ninguna caracteristica del piston (carrera, longitud, modelo) interviene.
%
%   ENTRADAS
%     alpha : roll  [rad]  giro alrededor de x
%     theta : pitch [rad]  giro alrededor de y
%     z     : [m]  separacion vertical COMANDADA entre el plano de anclaje
%                  del SORPOTE (abajo) y el del TRIANGULO (arriba).
%                  En la pose ensamblada vale Z0.
%
%   SALIDAS
%     dL : 3x1 [m]  ESTA es la que va a los Prismatic Joint. Desplazamiento
%                   respecto de la pose ensamblada del CAD. Vale [0;0;0]
%                   exactamente cuando alpha=theta=0 y z=Z0.
%     L  : 3x1 [m]  distancia entre centros de rotula (diagnostico).
%     L0 : 1x1 [m]  distancia nominal, DERIVADA de la geometria.
%
%   ORDEN: indice 1 <-> F1 (phi=-30), 2 <-> F2 (phi=90), 3 <-> F3 (phi=210),
%   el mismo de las columnas de T en Script_MARLUP_Final.m.
%
%   Modelo:  T_0^P = Trasl(0,0,z) * Ry(theta) * Rx(alpha)
%            L_i   = || T_0^P * p_i^P  -  b_i ||
%#codegen

% ============ UNICOS PARAMETROS: medirlos en el ensamblaje CAD ===========
R_BASE = 0.7608;   % [m] radio del anclaje inferior (SORPOTE), eje -> centro rotula
%R_TOP  = 0.143;   % [m] radio del anclaje superior (TRIANGULO), idem
Z0     = 1.377;   % [m] separacion vertical entre ambos planos, pose ensamblada
% =========================================================================

PHI = [-30; 90; 210] * pi/180;      % distribucion angular de los tres brazos

DR = R_BASE - R_TOP;
L0 = sqrt(DR*DR + Z0*Z0);           % longitud nominal: RESULTADO, no dato

ca = cos(alpha);  sa = sin(alpha);
ct = cos(theta);  st = sin(theta);

R = [  ct,  sa*st,  ca*st ;         % Ry(theta)*Rx(alpha)
        0,     ca,    -sa ;
      -st,  sa*ct,  ca*ct ];

L = zeros(3,1);
for i = 1:3
    cp = cos(PHI(i));
    sp = sin(PHI(i));

    b  = [R_BASE*cp; R_BASE*sp; 0];   % anclaje inferior, fijo en la base
    pP = [R_TOP*cp;  R_TOP*sp;  0];   % anclaje superior, en el marco movil
    d  = R*pP + [0; 0; z] - b;

    L(i) = sqrt(d(1)*d(1) + d(2)*d(2) + d(3)*d(3));
end

dL = L - L0;
end
